simulink model "lab2_simulink"  (R2025b)
settings: Solver=ode4  StartTime=0.0  StopTime=30  FixedStep=0.01  RelTol=1e-3
settings Model: Creator=golub  LastModifiedBy=golub

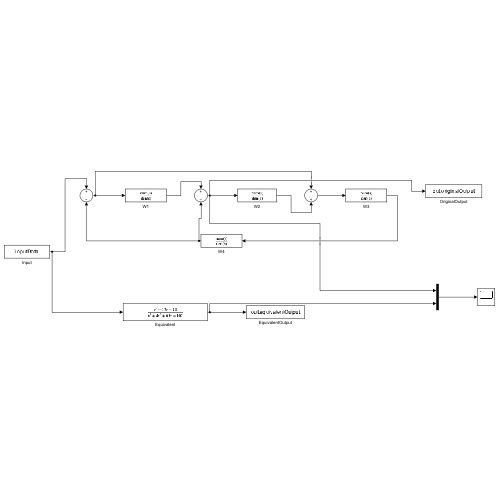
[thumbnail: Simulink's stored preview of the top-level diagram]
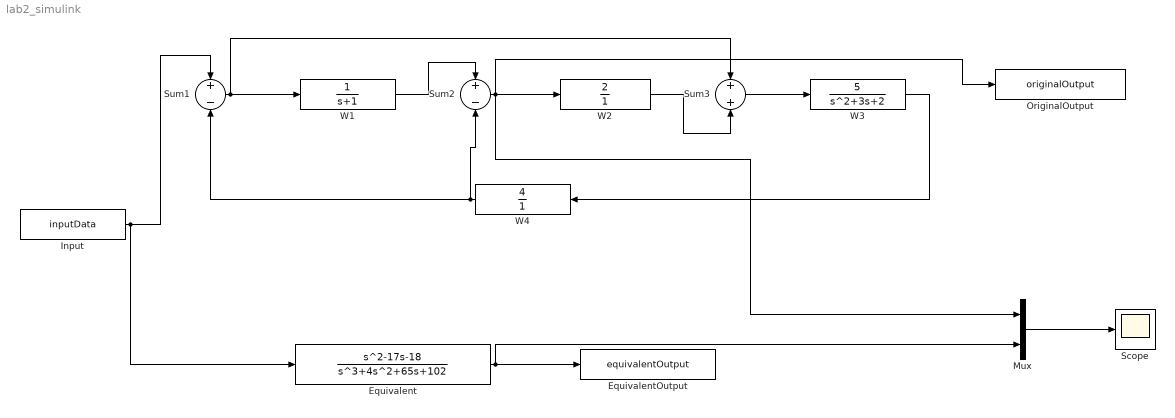
== system lab2_simulink ==
  Equivalent : TransferFcn  Numerator=[1 -17 -18]  Denominator=[1 4 65 102]
  EquivalentOutput : ToWorkspace  VariableName=equivalentOutput  SaveFormat=Timeseries  SampleTime=-1
  Input : FromWorkspace  VariableName=inputData  Interpolate=off  OutputAfterFinalValue=Holding final value
  Mux : Mux  Inputs=2
  OriginalOutput : ToWorkspace  VariableName=originalOutput  SaveFormat=Timeseries  SampleTime=-1
  Scope : Scope
      settings: ActiveDisplayYMinimum=-0.498419023115045  ActiveDisplayYMaximum=0.08214605876469587
  Sum1 : Sum  Inputs=+-
  Sum2 : Sum  Inputs=+-
  Sum3 : Sum
  W1 : TransferFcn  Numerator=1  Denominator=[1 1]
  W2 : TransferFcn  Numerator=2  Denominator=1
  W3 : TransferFcn  Numerator=5  Denominator=[1 3 2]
  W4 : TransferFcn  Numerator=4  Denominator=1
  wires:
  Input/1 -> Sum1/1, Equivalent/1
  Sum1/1 -> W1/1, Sum3/1
  W1/1 -> Sum2/1
  Sum2/1 -> W2/1, OriginalOutput/1, Mux/1
  W2/1 -> Sum3/2
  Sum3/1 -> W3/1
  W3/1 -> W4/1
  W4/1 -> Sum1/2, Sum2/2
  Equivalent/1 -> EquivalentOutput/1, Mux/2
  Mux/1 -> Scope/1
